simulink model "ParrotMinidroneKeyboardControl"  (R2025b)
settings: Solver=ode3  StartTime=0  StopTime=TFinal  FixedStep=Ts  RelTol=1e-3  EnableMultiTasking=on
values from neighbouring files (symbols this model uses):
  sensorCalibrationData = [0.09 -0.06 -9.473 -0.0095 -0.0075 0.0015 101270.95 0.2]    [sensorCalibration.mat]
undefined symbols (not defined in the file or in its folder): Command, ft, gcbh, init, m, Rec, s, SDTV, Sensors, States, stop_time, takeOffDuration, Ts, Vehicle, vrmfunc, VTs
libraries: simulink x16, aerolibconvert2 x4, SignalEditorBlockLib x2, environmentLibrary x2, visionconversions x2, visiongeotforms x2, aerolibutil x2, aerolibanimutils x1, aerolibnav x1, vrlib x1
(part 1 of 2)
settings Model: ModifiedByFormat=Krishna vamshi challa  ExtModeTrigDuration=80  Creator=The MathWorks, Inc.  LastModifiedBy=Krishna vamshi challa
settings SolverCC: AlgebraicLoopSolver=TrustRegion
settings DataIOCC: LimitDataPoints=on  SaveFormat=Array
settings OptimizationCC: BlockReduction=off  DefaultParameterBehavior=Inlined  EnhancedBackFolding=on  PassReuseOutputArgsAs=Individual arguments  ZeroExternalMemoryAtStartup=off  ZeroInternalMemoryAtStartup=off  MaxStackSize=64  OptimizeBlockOrder=speed  DifferentSizesBufferReuse=on  OptimizationCustomize=off  EfficientTunableParamExpr=on
settings DebuggingCC: AlgebraicLoopMsg=none  ParameterPrecisionLossMsg=none  ParameterTunabilityLossMsg=error  AllowSymbolicDim=off  PregeneratedLibrarySubsystemCodeDiagnostic=none  SubsystemReferenceDiagnosticForUnitTest=warning  SFUnexpectedBacktrackingDiag=warning  SFNoUnconditionalDefaultTransitionDiag=warning  SFExecutionAtInitializationDiag=none  ArithmeticOperatorsInVariantConditions=warning
settings HardwareCC: ProdBitPerPointer=32.0  ProdBitPerSizeT=32.0  ProdBitPerPtrDiffT=32.0  ProdLargestAtomicInteger=Long  ProdWordSize=32.0  ProdHWDeviceType=ARM Compatible->ARM 9
settings ModelReferenceCC: EnableRefExpFcnMdlSchedulingChecks=on  PropagateSignalLabelsOutOfModel=off
settings SFSimCC: SimUseLocalCustomCode=off  MATLABDynamicMemAlloc=off
settings RTWCC: SystemTargetFile=ert.tlc  HardwareBoard=PARROT Mambo  TemplateMakefile=ert_default_tmf  GenerateReport=on  RTWUseLocalCustomCode=off  Toolchain=Sourcery G++ Lite GNU Toolchain for Drones  LaunchReport=on  TargetLang=C++  GPUComputeCapability=3.5  Description=Embedded Coder
settings CodeAppCC: ForceParamTrailComments=on  IgnoreCustomStorageClasses=off  OperatorAnnotations=on  SimulinkDataObjDesc=on  SFDataObjDesc=on  InsertBlockDesc=on
settings ERTTargetCC: ExtModeMaxTrigDuration=80.0  RootIOFormat=Structure reference  TargetLangStandard=C++11 (ISO)  CodeInterfacePackaging=C++ class  SubcomponentCodeInterfacePackaging=C++ class
settings ConfigComp: CovMetricSettings=dw  CovSaveCumulativeToWorkspaceVar=on  CovSaveSingleToWorkspaceVar=on  CovExternalEMLEnable=off  CovSFcnEnable=off

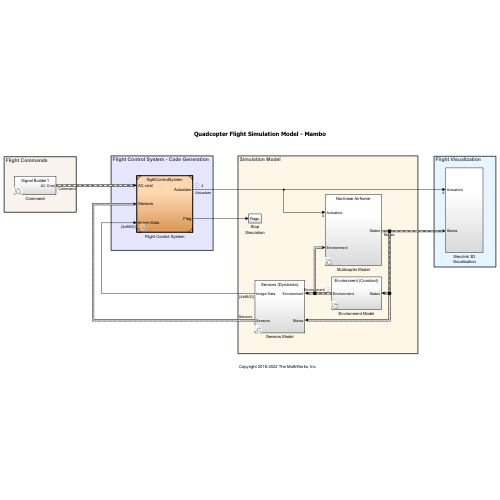
[thumbnail: Simulink's stored preview of the top-level diagram]
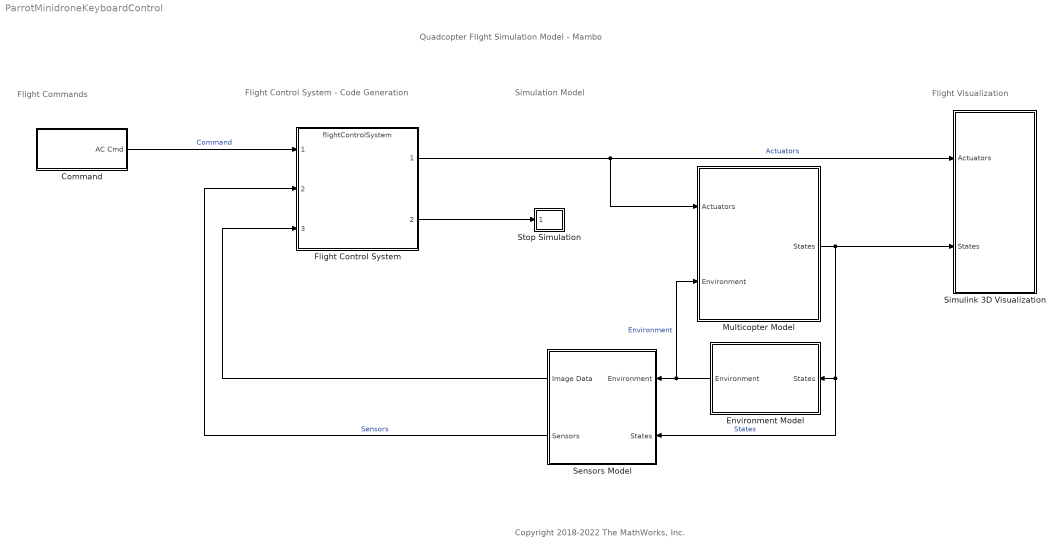
== system ParrotMinidroneKeyboardControl ==
  note: Flight Visualization
  note: Simulation Model
  note: Flight Control System - Code Generation
  note: Flight Commands
  note: Quadcopter Flight Simulation Model - Mambo
  note: Copyright 2018-2022 The MathWorks, Inc.
  Command : Subsystem  Variant=on
  Environment Model : Subsystem  Variant=on
  Flight Control System : ModelReference  ModelNameDialog=flightControlSystem.slx  SimulationMode=Normal  ModelReferenceVersion=11.6
  Multicopter Model : Subsystem  Variant=on
  Sensors Model : Subsystem  Variant=on
  Simulink 3D Visualization : Subsystem
  Stop Simulation : Subsystem
  wires:
  Command/1(AC Cmd) -> Flight Control System/1  "Command"
  Sensors Model/2(Sensors) -> Flight Control System/2  "Sensors"
  Flight Control System/1 -> Multicopter Model/1(Actuators), Simulink 3D Visualization/1(Actuators)  "Actuators"
  Environment Model/1(Environment) -> Sensors Model/1(Environment), Multicopter Model/2(Environment)  "Environment"
  Multicopter Model/1(States) -> Sensors Model/2(States), Environment Model/1(States), Simulink 3D Visualization/2(States)  "States"
  Flight Control System/2 -> Stop Simulation/1(Flags)
  Sensors Model/1(Image Data) -> Flight Control System/3

== system ParrotMinidroneKeyboardControl/Command ==
  note: VSS_COMMAND = 0 will select Signal Builder
      | VSS_COMMAND =1 will select Joystick + Signal Builder
      | VSS_COMMAND = 2 will select pre-saved data from .mat file
      | VSS_COMMAND = 3 will select pre-saved data from a spreadsheet
  Data : Subsystem  VariantControl=VSS_COMMAND_PRESAVED
  Joystick : Subsystem  VariantControl=VSS_COMMAND_JOYSTICK
  Signal Builder1 : Subsystem  VariantControl=VSS_COMMAND_SIGBLDR
  Spreadsheet Data : Subsystem  VariantControl=VSS_COMMAND_SPREADSHEET
  AC Cmd : Outport  OutDataTypeStr=Bus: CommandBus  VectorParamsAs1DForOutWhenUnconnected=off

== system ParrotMinidroneKeyboardControl/Environment Model ==
  note: VSS_ENVIRONMENT = 0 will select constant environment variables
      | VSS_ENVIRONMENT = 1 will select environment variables depending on position
  States : Inport  OutDataTypeStr=Bus: StatesBus
  Environment (Constant) : environmentLibrary/Environment (Constant)  SystemSampleTime=-1  VariantControl=VSS_ENVIRONMENT_CST  VariantActivationTime=update diagram  EmptyChoice=off  PassThrough=off  PassThroughVariantControl=(default)  EmptyChoiceVariantControl=(default)  AllowFlexibleInterface=on  Latency=0  AutoFrameSizeCalculation=off
  Environment (Variable) : environmentLibrary/Environment (Variable)  SystemSampleTime=-1  VariantControl=VSS_ENVIRONMENT_VARIABLE  VariantActivationTime=update diagram  AllowFlexibleInterface=on  Latency=0  AutoFrameSizeCalculation=off
  Environment : Outport  OutDataTypeStr=Bus: EnvironmentBus  VectorParamsAs1DForOutWhenUnconnected=off

== system ParrotMinidroneKeyboardControl/Multicopter Model ==
  note: VSS_VEHICLE = 0 will select linear airframe
      | VSS_VEHICLE = 1 will select nonlnear airframe
  Actuators : Inport
  Environment : Inport  Port=2  OutDataTypeStr=Bus: EnvironmentBus
  Linear Airframe : ModelReference  ModelNameDialog=linearAirframe.slx  SimulationMode=Normal  VariantControl=VSS_VEHICLE_LINEAR  ModelReferenceVersion=10.0
  Nonlinear Airframe : ModelReference  ModelNameDialog=nonlinearAirframe.slx  SimulationMode=Normal  VariantControl=VSS_VEHICLE_NONLINEAR  ModelReferenceVersion=12.2
  States : Outport  OutDataTypeStr=Bus: StatesBus  VectorParamsAs1DForOutWhenUnconnected=off

== system ParrotMinidroneKeyboardControl/Sensors Model ==
  note: VSS_SENSORS = 0 will select feedthrough sensors
      | VSS_SENSORS = 1 will select dynamics sensors with noise
  Environment : Inport
  States : Inport  Port=2
  Sensors (Dynamics) : Subsystem  TreatAsAtomicUnit=on  VariantControl=VSS_SENSORS_DYNAMICS
  Sensors (Feedthrough) : Subsystem  TreatAsAtomicUnit=on  VariantControl=VSS_SENSORS_FEEDTHROUGH
  Image Data : Outport  VectorParamsAs1DForOutWhenUnconnected=off
  Sensors : Outport  Port=2  VectorParamsAs1DForOutWhenUnconnected=off

== system ParrotMinidroneKeyboardControl/Simulink 3D Visualization ==
  Actuators : Inport
  States : Inport  Port=2
  Airspeed Indicator : AirspeedIndicatorBlock  LabelPosition=Hide
  Altimeter : AltimeterBlock  LabelPosition=Hide
  Artificial Horizon : ArtificialHorizonBlock  LabelPosition=Hide
  Climb Rate Indicator : ClimbIndicatorBlock  LabelPosition=Hide
  Extract Flight Instruments : Subsystem
  Heading Indicator1 : HeadingIndicatorBlock  LabelPosition=Hide
  Simulink 3D : Subsystem  VariantControl=VSS_VISUALIZATION_SL3D
      mask init:
      | visualizationFlightGearVars;
  Thruster {1..4} (4 alike) : RPMIndicatorBlock  LabelPosition=Hide
  wires:
  Actuators/1 -> Extract Flight Instruments/1(Actuators), Simulink 3D/2(Actuators)
  States/1 -> Extract Flight Instruments/2(States), Simulink 3D/1(States)

== system ParrotMinidroneKeyboardControl/Stop Simulation ==
  Flags : Inport  OutDataTypeStr=uint8
  Compare To Zero : simulink/Logic and Bit Operations/Compare To Zero  relop=>  OutDataTypeStr=boolean
  Flag has been triggered : Assertion
  Logical Operator : Logic  Operator=NOT  AllPortsSameDT=off  OutDataTypeStr=boolean
  wires:
  Flags/1 -> Compare To Zero/1
  Logical Operator/1 -> Flag has been triggered/1
  Compare To Zero/1 -> Logical Operator/1

== system ParrotMinidroneKeyboardControl/Command/Data ==
  Bus Creator : BusCreator  Inputs=5  OutDataTypeStr=Bus: CommandBus  NonVirtualBus=on
  Clock : Clock
  Compare To Constant : simulink/Logic and Bit Operations/Compare To Constant  relop=<  const=takeOffDuration  OutDataTypeStr=boolean
  Compare To Zero : simulink/Logic and Bit Operations/Compare To Zero  relop===  OutDataTypeStr=boolean
  Compare To Zero1 : simulink/Logic and Bit Operations/Compare To Zero  relop===  OutDataTypeStr=boolean
  Data Type Conversion1 : DataTypeConversion  OutDataTypeStr=single  SaturateOnIntegerOverflow=off  RndMeth=Floor
  Data Type Conversion3 : DataTypeConversion  OutDataTypeStr=single  SaturateOnIntegerOverflow=off  RndMeth=Floor
  Demux : Demux  Outputs=6
  From File : FromFile  FileName=cmdData.mat  SampleTime=Ts
  Live Time Ticks : simulink/Sources/Counter Free-Running  NumBits=32  tsamp=Ts
  Logical Operator : Logic  AllPortsSameDT=off  OutDataTypeStr=boolean
  Mux : Mux  Inputs=3
  Mux1 : Mux  Inputs=3
  Rate Transition{1..4} (4 alike) : RateTransition  OutPortSampleTime=Ts
  AC Cmd : Outport  OutDataTypeStr=Bus: CommandBus  VectorParamsAs1DForOutWhenUnconnected=off
  wires:
  Demux/4 -> Mux/1  "roll_cmd"
  Demux/5 -> Mux/2, Compare To Zero1/1  "pitch_cmd"
  Demux/6 -> Compare To Zero/1, Mux/3  "yaw_cmd"
  From File/1 -> Demux/1
  Logical Operator/1 -> Rate Transition4/1
  Rate Transition1/1 -> Bus Creator/4  "orient_ref"
  Rate Transition2/1 -> Bus Creator/2  "pos_ref"
  Demux/3 -> Mux1/3
  Mux/1 -> Data Type Conversion3/1
  Data Type Conversion1/1 -> Rate Transition2/1
  Demux/1 -> Mux1/1
  Compare To Zero1/1 -> Logical Operator/2
  Compare To Zero/1 -> Logical Operator/1
  Mux1/1 -> Data Type Conversion1/1
  Clock/1 -> Compare To Constant/1
  Rate Transition4/1 -> Bus Creator/1  "controlModePosVSOrient"
  Data Type Conversion3/1 -> Rate Transition1/1
  Demux/2 -> Mux1/2
  Compare To Constant/1 -> Rate Transition3/1
  Rate Transition3/1 -> Bus Creator/3  "takeoff_flag"
  Live Time Ticks/1 -> Bus Creator/5  "live_time_ticks"
  Bus Creator/1 -> AC Cmd/1

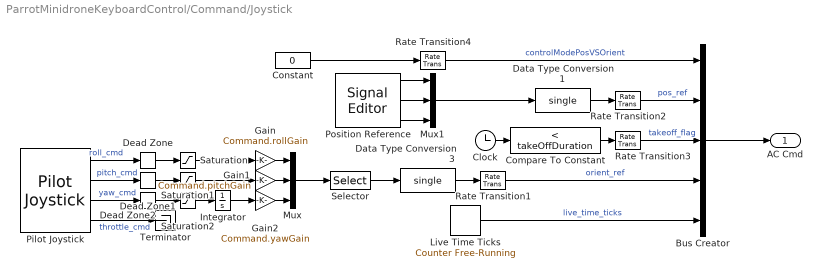
== system ParrotMinidroneKeyboardControl/Command/Joystick ==
  Bus Creator : BusCreator  Inputs=5  OutDataTypeStr=Bus: CommandBus  NonVirtualBus=on
  Clock : Clock
  Compare To Constant : simulink/Logic and Bit Operations/Compare To Constant  relop=<  const=takeOffDuration  OutDataTypeStr=boolean
  Constant : Constant  Value=0  OutDataTypeStr=boolean
  Data Type Conversion1 : DataTypeConversion  OutDataTypeStr=single  SaturateOnIntegerOverflow=off  RndMeth=Floor
  Data Type Conversion3 : DataTypeConversion  OutDataTypeStr=single  SaturateOnIntegerOverflow=off  RndMeth=Floor
  Dead Zone : DeadZone  LowerValue=Command.rollDeadZoneStart  UpperValue=Command.rollDeadZoneEnd
  Dead Zone1 : DeadZone  LowerValue=Command.pitchDeadZoneStart  UpperValue=Command.pitchDeadZoneEnd
  Dead Zone2 : DeadZone  LowerValue=Command.yawDeadZoneStart  UpperValue=Command.yawDeadZoneEnd
  Gain : Gain  Gain=Command.rollGain
  Gain1 : Gain  Gain=Command.pitchGain
  Gain2 : Gain  Gain=Command.yawGain
  Integrator : Integrator
  Live Time Ticks : simulink/Sources/Counter Free-Running  NumBits=32  tsamp=Ts
  Mux : Mux  Inputs=3
  Mux1 : Mux  Inputs=3
  Pilot Joystick : aerolibanimutils/Pilot Joystick  JoystickID=Joystick1  OutputConfiguration=FourAxis  SampleTime=Ts
  Position Reference : SignalEditorBlockLib/Signal Editor  FileName=Position_Reference.mat  ActiveScenario=Group_1  ActiveSignal=Z  IsBus=off  OutputBusObjectStr=Bus: BusObject  SampleTime=0  OutputAfterFinalValue=Extrapolation  Unit=inherit  PreserveSignalName=on  ApplySigPropsToAllScenarios=on  ApplySigPropsToAllSignals=off
  Rate Transition{1..4} (4 alike) : RateTransition  OutPortSampleTime=Ts
  Saturation : Saturate  UpperLimit=Command.rollSatUpper  LowerLimit=Command.rollSatLower
  Saturation1 : Saturate  UpperLimit=Command.pitchSatUpper  LowerLimit=Command.pitchSatLower
  Saturation2 : Saturate  UpperLimit=Command.yawSatUpper  LowerLimit=Command.yawSatLower
  Selector : Selector  InputPortWidth=3  IndexOptions=Index vector (dialog)  Indices=[3 2 1]  OutputSizes=1
  Terminator : Terminator
  AC Cmd : Outport  OutDataTypeStr=Bus: CommandBus  VectorParamsAs1DForOutWhenUnconnected=off
  wires:
  Pilot Joystick/4 -> Terminator/1  "throttle_cmd"
  Pilot Joystick/1 -> Dead Zone/1  "roll_cmd"
  Bus Creator/1 -> AC Cmd/1
  Constant/1 -> Rate Transition4/1
  Rate Transition1/1 -> Bus Creator/4  "orient_ref"
  Rate Transition2/1 -> Bus Creator/2  "pos_ref"
  Position Reference/3 -> Mux1/3
  Mux/1 -> Selector/1
  Data Type Conversion1/1 -> Rate Transition2/1
  Position Reference/1 -> Mux1/1
  Mux1/1 -> Data Type Conversion1/1
  Compare To Constant/1 -> Rate Transition3/1
  Clock/1 -> Compare To Constant/1
  Rate Transition4/1 -> Bus Creator/1  "controlModePosVSOrient"
  Data Type Conversion3/1 -> Rate Transition1/1
  Pilot Joystick/2 -> Dead Zone1/1  "pitch_cmd"
  Position Reference/2 -> Mux1/2
  Rate Transition3/1 -> Bus Creator/3  "takeoff_flag"
  Live Time Ticks/1 -> Bus Creator/5  "live_time_ticks"
  Selector/1 -> Data Type Conversion3/1
  Dead Zone/1 -> Saturation/1
  Saturation/1 -> Gain/1
  Gain/1 -> Mux/1
  Dead Zone1/1 -> Saturation1/1
  Saturation1/1 -> Gain1/1
  Gain1/1 -> Mux/2
  Dead Zone2/1 -> Saturation2/1
  Saturation2/1 -> Integrator/1
  Gain2/1 -> Mux/3
  Pilot Joystick/3 -> Dead Zone2/1  "yaw_cmd"
  Integrator/1 -> Gain2/1

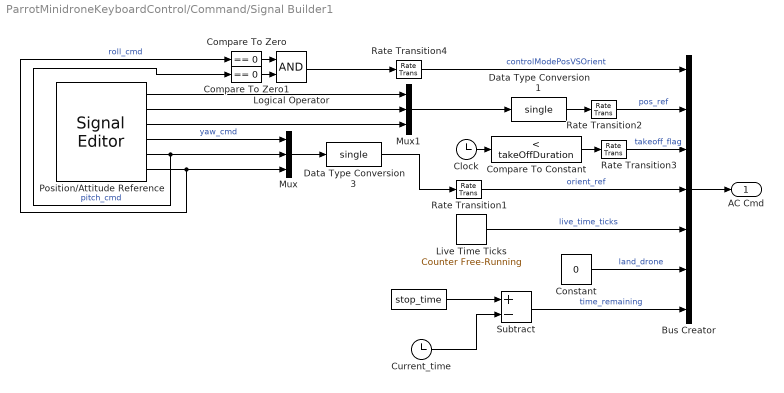
== system ParrotMinidroneKeyboardControl/Command/Signal Builder1 ==
  " " : Constant  InitFcn=|  Value=stop_time
      | sim_model = split(gcs,"/");
      | stop_time_str = get_param(sim_model{1},'stopTime');
      | stop_time = evalin('base', stop_time_str);
      settings: DeleteFcn=clear sim_model stop_time_str stop_time
  Bus Creator : BusCreator  Inputs=7  OutDataTypeStr=Bus: CommandBus  NonVirtualBus=on
  Clock : Clock
  Compare To Constant : simulink/Logic and Bit Operations/Compare To Constant  relop=<  const=takeOffDuration  OutDataTypeStr=boolean
  Compare To Zero : simulink/Logic and Bit Operations/Compare To Zero  relop===  OutDataTypeStr=boolean
  Compare To Zero1 : simulink/Logic and Bit Operations/Compare To Zero  relop===  OutDataTypeStr=boolean
  Constant : Constant  Value=0  OutDataTypeStr=boolean
  Current_time : Clock
  Data Type Conversion1 : DataTypeConversion  OutDataTypeStr=single  SaturateOnIntegerOverflow=off  RndMeth=Floor
  Data Type Conversion3 : DataTypeConversion  OutDataTypeStr=single  SaturateOnIntegerOverflow=off  RndMeth=Floor
  Live Time Ticks : simulink/Sources/Counter Free-Running  NumBits=32  tsamp=Ts
  Logical Operator : Logic  AllPortsSameDT=off  OutDataTypeStr=boolean
  Mux : Mux  Inputs=3
  Mux1 : Mux  Inputs=3
  Position/Attitude Reference : SignalEditorBlockLib/Signal Editor  FileName=Position_Attitude_Reference.mat  ActiveScenario=Group_1  ActiveSignal=Roll  IsBus=off  OutputBusObjectStr=Bus: BusObject  SampleTime=0  OutputAfterFinalValue=Extrapolation  Unit=inherit  PreserveSignalName=on  ApplySigPropsToAllScenarios=on  ApplySigPropsToAllSignals=off  SignalPropertySource=Dialog parameters
  Rate Transition{1..4} (4 alike) : RateTransition  OutPortSampleTime=Ts
  Subtract : Sum  Inputs=+-
  AC Cmd : Outport  OutDataTypeStr=Bus: CommandBus  VectorParamsAs1DForOutWhenUnconnected=off
  wires:
  Bus Creator/1 -> AC Cmd/1
  Position/Attitude Reference/6 -> Compare To Zero/1, Mux/3  "roll_cmd"
  Position/Attitude Reference/5 -> Mux/2, Compare To Zero1/1  "pitch_cmd"
  Position/Attitude Reference/4 -> Mux/1  "yaw_cmd"
  Mux/1 -> Data Type Conversion3/1
  Data Type Conversion3/1 -> Rate Transition1/1
  Rate Transition1/1 -> Bus Creator/4  "orient_ref"
  Compare To Zero/1 -> Logical Operator/1
  Compare To Zero1/1 -> Logical Operator/2
  Logical Operator/1 -> Rate Transition4/1
  Rate Transition4/1 -> Bus Creator/1  "controlModePosVSOrient"
  Position/Attitude Reference/1 -> Mux1/1
  Position/Attitude Reference/2 -> Mux1/2
  Position/Attitude Reference/3 -> Mux1/3
  Mux1/1 -> Data Type Conversion1/1
  Data Type Conversion1/1 -> Rate Transition2/1
  Rate Transition2/1 -> Bus Creator/2  "pos_ref"
  Clock/1 -> Compare To Constant/1
  Compare To Constant/1 -> Rate Transition3/1
  Rate Transition3/1 -> Bus Creator/3  "takeoff_flag"
  Live Time Ticks/1 -> Bus Creator/5  "live_time_ticks"
  Constant/1 -> Bus Creator/6  "land_drone"
  Subtract/1 -> Bus Creator/7  "time_remaining"
  Current_time/1 -> Subtract/2
  " "/1 -> Subtract/1

== system ParrotMinidroneKeyboardControl/Command/Spreadsheet Data ==
  Bus Creator : BusCreator  Inputs=5  OutDataTypeStr=Bus: CommandBus  NonVirtualBus=on
  Clock : Clock
  Compare To Constant : simulink/Logic and Bit Operations/Compare To Constant  relop=<  const=takeOffDuration  OutDataTypeStr=boolean
  Compare To Zero : simulink/Logic and Bit Operations/Compare To Zero  relop===  OutDataTypeStr=boolean
  Compare To Zero1 : simulink/Logic and Bit Operations/Compare To Zero  relop===  OutDataTypeStr=boolean
  Data Type Conversion1 : DataTypeConversion  OutDataTypeStr=single  SaturateOnIntegerOverflow=off  RndMeth=Floor
  Data Type Conversion3 : DataTypeConversion  OutDataTypeStr=single  SaturateOnIntegerOverflow=off  RndMeth=Floor
  From Spreadsheet : FromSpreadsheet  FileName=cmdData.xlsx  SheetName=data  SampleTime=Ts
  Live Time Ticks : simulink/Sources/Counter Free-Running  NumBits=32  tsamp=Ts
  Logical Operator : Logic  AllPortsSameDT=off  OutDataTypeStr=boolean
  Mux : Mux  Inputs=3
  Mux1 : Mux  Inputs=3
  Rate Transition{1..4} (4 alike) : RateTransition  OutPortSampleTime=Ts
  AC Cmd : Outport  OutDataTypeStr=Bus: CommandBus  VectorParamsAs1DForOutWhenUnconnected=off
  wires:
  Bus Creator/1 -> AC Cmd/1
  From Spreadsheet/4 -> Mux/1  "roll_cmd"
  From Spreadsheet/6 -> Mux/3, Compare To Zero/1  "yaw_cmd"
  Logical Operator/1 -> Rate Transition4/1
  Rate Transition1/1 -> Bus Creator/4  "orient_ref"
  Rate Transition2/1 -> Bus Creator/2  "pos_ref"
  From Spreadsheet/3 -> Mux1/3
  Mux/1 -> Data Type Conversion3/1
  Data Type Conversion1/1 -> Rate Transition2/1
  From Spreadsheet/1 -> Mux1/1
  Compare To Zero1/1 -> Logical Operator/2
  Compare To Zero/1 -> Logical Operator/1
  Mux1/1 -> Data Type Conversion1/1
  Compare To Constant/1 -> Rate Transition3/1
  Clock/1 -> Compare To Constant/1
  Rate Transition4/1 -> Bus Creator/1  "controlModePosVSOrient"
  Data Type Conversion3/1 -> Rate Transition1/1
  From Spreadsheet/5 -> Mux/2, Compare To Zero1/1  "pitch_cmd"
  From Spreadsheet/2 -> Mux1/2
  Rate Transition3/1 -> Bus Creator/3  "takeoff_flag"
  Live Time Ticks/1 -> Bus Creator/5  "live_time_ticks"

== system ParrotMinidroneKeyboardControl/Sensors Model/Sensors (Dynamics) ==
  States : Inport  OutDataTypeStr=Bus: StatesBus
  Environment : Inport  Port=2  OutDataTypeStr=Bus: EnvironmentBus
  Bus Creator1 : BusCreator  Inputs=3  OutDataTypeStr=Bus: SensorsBus  NonVirtualBus=on
  Bus Creator2 : BusCreator  Inputs=3  OutDataTypeStr=Bus: extraSensorData_t  NonVirtualBus=on
  Constant : Constant  Value=sensorCalibrationData  OutDataTypeStr=single
  Memory1 : Memory  InitialCondition=States  InheritSampleTime=on
  Sensor System : Subsystem
  _DUMMY_FLAG_usePosVIS : Constant  Value=Sensors.dummy.usePosVISFlag  OutDataTypeStr=single  SampleTime=Ts
  _DUMMY_posVIS : Constant  Value=Sensors.dummy.posVISNoVisionAvail  OutDataTypeStr=single  SampleTime=Ts
  Sensors : Outport  OutDataTypeStr=Bus: SensorsBus  VectorParamsAs1DForOutWhenUnconnected=off
  Image Data : Outport  Port=2  VectorParamsAs1DForOutWhenUnconnected=off
  wires:
  Constant/1 -> Bus Creator1/3  "SensorCalibration"
  Memory1/1 -> Sensor System/1(States)
  Bus Creator2/1 -> Bus Creator1/1  "VisionSensors"
  Bus Creator1/1 -> Sensors/1
  States/1 -> Memory1/1
  Environment/1 -> Sensor System/2(Environment)
  _DUMMY_FLAG_usePosVIS/1 -> Bus Creator2/3  "usePosVIS_flag"
  _DUMMY_posVIS/1 -> Bus Creator2/2  "posVIS_data"
  Sensor System/1(opticalFlow_data) -> Bus Creator2/1  "opticalFlow_data"
  Sensor System/2(sensordata_data) -> Bus Creator1/2  "HALSensors"
  Sensor System/3(camera_data) -> Image Data/1

== system ParrotMinidroneKeyboardControl/Sensors Model/Sensors (Feedthrough) ==
  States : Inport  OutDataTypeStr=Bus: StatesBus
  Environment : Inport  Port=2  OutDataTypeStr=Bus: EnvironmentBus
  Bus Creator1 : BusCreator  Inputs=3  OutDataTypeStr=Bus: SensorsBus  NonVirtualBus=on
  Bus Creator2 : BusCreator  Inputs=3  OutDataTypeStr=Bus: extraSensorData_t  NonVirtualBus=on
  Constant1 : Constant  Value=sensorCalibrationData  OutDataTypeStr=single
  Memory : Memory  InitialCondition=States  InheritSampleTime=on
  Sensor System : Subsystem
  _DUMMY_FLAG_usePosVIS : Constant  Value=Sensors.dummy.usePosVISFlag  OutDataTypeStr=single
  _DUMMY_posVIS : Constant  Value=Sensors.dummy.posVISNoVisionAvail  OutDataTypeStr=single
  Sensors : Outport  OutDataTypeStr=Bus: SensorsBus  VectorParamsAs1DForOutWhenUnconnected=off
  Image Data : Outport  Port=2  VectorParamsAs1DForOutWhenUnconnected=off
  wires:
  Constant1/1 -> Bus Creator1/3  "SensorCalibration"
  Memory/1 -> Sensor System/1(States)
  Sensor System/2(sensordata_data) -> Bus Creator1/2  "HALSensors"
  States/1 -> Memory/1
  Environment/1 -> Sensor System/2(Environment)
  Bus Creator1/1 -> Sensors/1
  _DUMMY_FLAG_usePosVIS/1 -> Bus Creator2/3  "usePosVIS_flag"
  Sensor System/1(opticalFlow_data) -> Bus Creator2/1  "opticalFlow_data"
  _DUMMY_posVIS/1 -> Bus Creator2/2  "posVIS_data"
  Bus Creator2/1 -> Bus Creator1/1  "VisionSensors"
  Sensor System/3(camera_data) -> Image Data/1

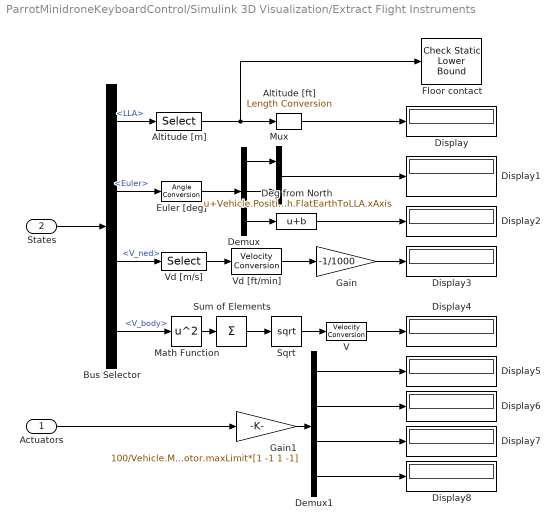
== system ParrotMinidroneKeyboardControl/Simulink 3D Visualization/Extract Flight Instruments ==
  Actuators : Inport
  States : Inport  Port=2
  Altitude [ft] : aerolibconvert2/Length Conversion  IU=m  OU=ft
  Altitude [m] : Selector  InputPortWidth=3  IndexOptions=Index vector (dialog)  Indices=[3]  OutputSizes=1
  Bus Selector : BusSelector  OutputSignals=LLA,Euler,V_ned,V_body
  Deg from North : Bias  Bias=Vehicle.PositionOnEarth.FlatEarthToLLA.xAxis  SaturateOnIntegerOverflow=off
  Demux : Demux  Outputs=3
  Demux1 : Demux
  Display{,1..8} (9 alike) : Display
  Euler [deg] : aerolibconvert2/Angle Conversion  IU=rad  OU=deg
  Floor contact : simulink/Model Verification/Check Static  Lower Bound  Description=init.posLLA(3) <= u  min=init.posLLA(3)  min_included=on  enabled=on  stopWhenAssertionFail=on  export=off  icon=graphic
  Gain : Gain  Gain=-1/1000
  Gain1 : Gain  Gain=100/Vehicle.Motor.maxLimit*[1 -1 1 -1]
  Math Function : Math  Operator=square  SignedPower=on
  Mux : Mux  Inputs=2
  Sqrt : Sqrt
  Sum of Elements : Sum  Inputs=+
  V : aerolibconvert2/Velocity Conversion  IU=m/s  OU=kts
  Vd [ft/min] : aerolibconvert2/Velocity Conversion  IU=m/s  OU=ft/min
  Vd [m/s] : Selector  InputPortWidth=3  IndexOptions=Index vector (dialog)  Indices=[3]  OutputSizes=1
  wires:
  Bus Selector/1 -> Altitude [m]/1  "<LLA>"
  Altitude [m]/1 -> Floor contact/1, Altitude [ft]/1
  States/1 -> Bus Selector/1
  Altitude [ft]/1 -> Display/1
  Bus Selector/2 -> Euler [deg]/1  "<Euler>"
  Euler [deg]/1 -> Demux/1
  Demux/1 -> Mux/1
  Demux/2 -> Mux/2
  Mux/1 -> Display1/1
  Deg from North/1 -> Display2/1
  Bus Selector/3 -> Vd [m/s]/1  "<V_ned>"
  Vd [m/s]/1 -> Vd [ft/min]/1
  Vd [ft/min]/1 -> Gain/1
  Gain/1 -> Display3/1
  Math Function/1 -> Sum of Elements/1
  Sum of Elements/1 -> Sqrt/1
  Bus Selector/4 -> Math Function/1  "<V_body>"
  Sqrt/1 -> V/1
  V/1 -> Display4/1
  Gain1/1 -> Demux1/1
  Demux1/1 -> Display5/1
  Demux1/2 -> Display6/1
  Demux1/3 -> Display7/1
  Demux1/4 -> Display8/1
  Actuators/1 -> Gain1/1
  Demux/3 -> Deg from North/1

== system ParrotMinidroneKeyboardControl/Simulink 3D Visualization/Simulink 3D ==
  States : Inport
  Actuators : Inport  Port=2
  Axes to VR Axes : Subsystem
  Axes to VR Axes Camera Chase : Subsystem
  Axes to VR Axes Camera Iso : Subsystem
  Bus Selector : BusSelector  OutputSignals=Euler,X_ned
  Camera bias Chase : Bias  Bias=[-4 0 -.9558]'  SaturateOnIntegerOverflow=off
  Camera bias Iso : Bias  Bias=[0.9009 .99 -.6247]'  SaturateOnIntegerOverflow=off
  Euler to VR : Subsystem
  Rate Transition{,1..3} (4 alike) : RateTransition
  Subsystem : Subsystem
  VR Sink : vrlib/VR Sink  InstantiateOnLoad=on  SampleTime=12*Ts  ViewEnable=on  RemoteChange=off  RemoteView=off  FieldsWritten=QuadBody.rotation.4.1.1.double#QuadBody.translation.3.1.1.double#Blade1.rotation.4.1.1.double#Blade3.rotation.4.1.1.double#Blade2.rotation.4.1.1.double#Blade4.rotation.4.1.1.double#IsoNoRotation.position.3.1.1.double#OnQuadNoRotation.position.3.1.1.double  WorldFileName=asbQuadcopterWorld.wrl  WorldDescription=Minidrone Flight Visualization  AutoView=on  VideoDimensions=[]  AllowVariableSize=off  FigureProperties="{'Position', 'Name', 'Viewpoint', 'CameraBound', 'CameraDirection', 'CameraPosition', 'CameraUpVector', 'ZoomFactor', 'Antialiasing', 'Headlight', 'Lighting', 'Sound', 'StatusBar', 'Stereo3D', 'Stereo3DCameraOffset', 'Stereo3DHIT', 'ToolBar', 'Textures', 'Transparency', 'Triad', 'Wireframe', 'NavZones', 'NavMode', 'NavSpeed', 'CaptureFileFormat', 'CaptureFileName', 'Record2DCompressMethod', 'Record2DCompressQuality', 'Record2D', 'Record2DFileName', 'Record2DFPS'; [5.0000000000000000e+00   9.2000000000000000e+01   5.7600000000000000e+02   3.8000000000000000e+02], 'Minidrone Flight Visualization', 'Isometric', 'on', [0.0000000000000000e+00   0.0000000000000000e+00  -1.0000000000000000e+00], [0.0000000000000000e+00   0.0000000000000000e+00   0.0000000000000000e+00], [0.0000000000000000e+00   1.0000000000000000e+00   0.0000000000000000e+00], [1.0000000000000000e+00], 'on', 'on', 'on', 'off', 'on', 'off', [1.0000000000000001e-01], [0.0000000000000000e+00], 'on', 'on', 'on', 'none', 'off', 'off', 'examine', 'normal', 'tif', '%f_anim_%n.tif', 'auto', [7.5000000000000000e+01], 'off', '%f_anim_%n.avi', 'auto'}"
  wires:
  Euler to VR/1(Axis Angle) -> Rate Transition/1
  Axes to VR Axes/1(Xe VR) -> Rate Transition1/1
  Bus Selector/1 -> Euler to VR/1(Euler Angles)  "<Euler>"
  Bus Selector/2 -> Camera bias Chase/1, Camera bias Iso/1, Axes to VR Axes/1(Xe)  "<X_ned>"
  States/1 -> Bus Selector/1
  Actuators/1 -> Subsystem/1(Actuators)
  Axes to VR Axes Camera Iso/1(Xe VR) -> Rate Transition2/1
  Camera bias Iso/1 -> Axes to VR Axes Camera Iso/1(Xe)
  Rate Transition/1 -> VR Sink/1
  Rate Transition1/1 -> VR Sink/2
  Subsystem/1(Position Blade1) -> VR Sink/3
  Subsystem/2(Position Blade 2) -> VR Sink/4
  Subsystem/3(Position Blade 3) -> VR Sink/5
  Subsystem/4(Position Blade 4) -> VR Sink/6
  Rate Transition2/1 -> VR Sink/7
  Axes to VR Axes Camera Chase/1(Xe VR) -> Rate Transition3/1
  Rate Transition3/1 -> VR Sink/8
  Camera bias Chase/1 -> Axes to VR Axes Camera Chase/1(Xe)

== system ParrotMinidroneKeyboardControl/Sensors Model/Sensors (Dynamics)/Sensor System ==
  States : Inport
  Environment : Inport  Port=2
  Camera : Subsystem
  IMU_Pressure : Subsystem
  Rate Transition1 : RateTransition  OutPortSampleTime=Ts
  Rate Transition2 : RateTransition  OutPortSampleTime=Ts
  opticalFlow_data : Outport  VectorParamsAs1DForOutWhenUnconnected=off
  sensordata_data : Outport  Port=2  OutDataTypeStr=Bus: HAL_acquisition_t  VectorParamsAs1DForOutWhenUnconnected=off
  camera_data : Outport  Port=3  VectorParamsAs1DForOutWhenUnconnected=off
  wires:
  Environment/1 -> IMU_Pressure/2(Environment)
  Camera/1(opticalFlow_datout) -> Rate Transition1/1
  IMU_Pressure/1(sensordata_datout) -> Rate Transition2/1
  Rate Transition1/1 -> opticalFlow_data/1
  Rate Transition2/1 -> sensordata_data/1
  States/1 -> Camera/1(states), IMU_Pressure/1(States)
  Camera/2(image_data) -> camera_data/1

== system ParrotMinidroneKeyboardControl/Sensors Model/Sensors (Feedthrough)/Sensor System ==
  States : Inport
  Environment : Inport  Port=2
  Camera : Subsystem
  IMU_Pressure : Subsystem
  Rate Transition1 : RateTransition  OutPortSampleTime=Ts
  Rate Transition2 : RateTransition  OutPortSampleTime=Ts
  opticalFlow_data : Outport  VectorParamsAs1DForOutWhenUnconnected=off
  sensordata_data : Outport  Port=2  OutDataTypeStr=Bus: HAL_acquisition_t  VectorParamsAs1DForOutWhenUnconnected=off
  camera_data : Outport  Port=3  VectorParamsAs1DForOutWhenUnconnected=off
  wires:
  Environment/1 -> IMU_Pressure/2(Environment)
  Camera/1(opticalFlow_datout) -> Rate Transition1/1
  IMU_Pressure/1(sensordata_datout) -> Rate Transition2/1
  Rate Transition1/1 -> opticalFlow_data/1
  Rate Transition2/1 -> sensordata_data/1
  States/1 -> Camera/1(states), IMU_Pressure/1(states_datin)
  Camera/2(image_data) -> camera_data/1

== system ParrotMinidroneKeyboardControl/Simulink 3D Visualization/Simulink 3D/Axes to VR Axes ==
  Xe : Inport
  Demux : Demux  Outputs=3
      settings: DisplayOption=none
  Mux : Mux  Inputs=3
  rad-->deg1 : Gain  Gain=-1  SaturateOnIntegerOverflow=on  OutDataTypeStr=Inherit: Same as input  ParamDataTypeStr=Inherit: Same as input
  Xe VR : Outport  VectorParamsAs1DForOutWhenUnconnected=off
  wires:
  Xe/1 -> Demux/1
  Demux/1 -> Mux/1
  Demux/3 -> rad-->deg1/1
  Mux/1 -> Xe VR/1
  rad-->deg1/1 -> Mux/2
  Demux/2 -> Mux/3

== system ParrotMinidroneKeyboardControl/Simulink 3D Visualization/Simulink 3D/Axes to VR Axes Camera Chase ==
  Xe : Inport
  Demux : Demux  Outputs=3
      settings: DisplayOption=none
  Mux : Mux  Inputs=3
  rad-->deg1 : Gain  Gain=-1  SaturateOnIntegerOverflow=on  OutDataTypeStr=Inherit: Same as input  ParamDataTypeStr=Inherit: Same as input
  Xe VR : Outport  VectorParamsAs1DForOutWhenUnconnected=off
  wires:
  Xe/1 -> Demux/1
  Demux/1 -> Mux/1
  Demux/3 -> rad-->deg1/1
  Mux/1 -> Xe VR/1
  rad-->deg1/1 -> Mux/2
  Demux/2 -> Mux/3

== system ParrotMinidroneKeyboardControl/Simulink 3D Visualization/Simulink 3D/Axes to VR Axes Camera Iso ==
  Xe : Inport
  Demux : Demux  Outputs=3
      settings: DisplayOption=none
  Mux : Mux  Inputs=3
  rad-->deg1 : Gain  Gain=-1  SaturateOnIntegerOverflow=on  OutDataTypeStr=Inherit: Same as input  ParamDataTypeStr=Inherit: Same as input
  Xe VR : Outport  VectorParamsAs1DForOutWhenUnconnected=off
  wires:
  Demux/2 -> Mux/3
  rad-->deg1/1 -> Mux/2
  Mux/1 -> Xe VR/1
  Demux/3 -> rad-->deg1/1
  Demux/1 -> Mux/1
  Xe/1 -> Demux/1

== system ParrotMinidroneKeyboardControl/Simulink 3D Visualization/Simulink 3D/Euler to VR ==
  Euler Angles : Inport
  Axis Angle Vector : Subsystem
  Mux : Mux  Inputs=2
  Mux1 : Mux  Inputs=2
  Mux2 : Mux  Inputs=2
  Quaternion Multiplication (Pitch & Yaw) : aerolibutil/Quaternion Multiplication
  Quaternion Multiplication (Roll) : aerolibutil/Quaternion Multiplication
  Quaternion Normalization : Subsystem
  Quaternion Normalization1 : Subsystem
  Quaternion Normalization2 : Subsystem
  Selector : Selector  InputPortWidth=3  IndexOptions=Index vector (dialog)  Indices=[3]  OutputSizes=1
  Selector1 : Selector  InputPortWidth=3  IndexOptions=Index vector (dialog)  Indices=[2]  OutputSizes=1
  Selector2 : Selector  InputPortWidth=3  IndexOptions=Index vector (dialog)  Indices=[1]  OutputSizes=1
  Vr Pitch Axes : Constant  Value=[0 0 1]
  Vr Roll Axes : Constant  Value=[1 0 0]
  Vr Yaw Axes : Constant  Value=[0 -1 0]
  Axis Angle : Outport  VectorParamsAs1DForOutWhenUnconnected=off
  wires:
  Quaternion Multiplication (Roll)/1 -> Axis Angle Vector/1(e0)
  Axis Angle Vector/1(e0_norm) -> Axis Angle/1
  Quaternion Normalization/1(e0_norm) -> Quaternion Multiplication (Roll)/2
  Quaternion Normalization2/1(e0_norm) -> Quaternion Multiplication (Pitch & Yaw)/1
  Quaternion Normalization1/1(e0_norm) -> Quaternion Multiplication (Pitch & Yaw)/2
  Mux2/1 -> Quaternion Normalization2/1(e0)
  Mux1/1 -> Quaternion Normalization1/1(e0)
  Mux/1 -> Quaternion Normalization/1(e0)
  Selector/1 -> Mux2/1
  Vr Yaw Axes/1 -> Mux2/2
  Selector1/1 -> Mux1/1
  Vr Pitch Axes/1 -> Mux1/2
  Selector2/1 -> Mux/1
  Vr Roll Axes/1 -> Mux/2
  Euler Angles/1 -> Selector2/1, Selector1/1, Selector/1
  Quaternion Multiplication (Pitch & Yaw)/1 -> Quaternion Multiplication (Roll)/1

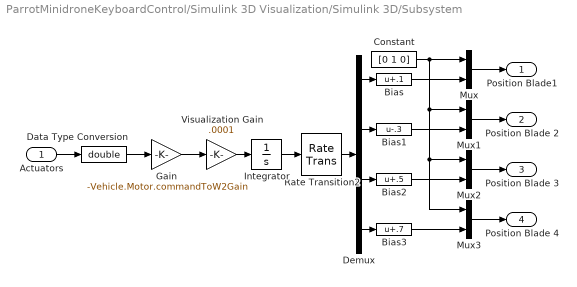
== system ParrotMinidroneKeyboardControl/Simulink 3D Visualization/Simulink 3D/Subsystem ==
  Actuators : Inport
  Bias : Bias  Bias=.1  SaturateOnIntegerOverflow=off
  Bias1 : Bias  Bias=-.3  SaturateOnIntegerOverflow=off
  Bias2 : Bias  Bias=.5  SaturateOnIntegerOverflow=off
  Bias3 : Bias  Bias=.7  SaturateOnIntegerOverflow=off
  Constant : Constant  Value=[0 1 0]
  Data Type Conversion : DataTypeConversion  OutDataTypeStr=double  SaturateOnIntegerOverflow=off  RndMeth=Floor
  Demux : Demux
  Gain : Gain  Gain=-Vehicle.Motor.commandToW2Gain
  Integrator : Integrator  InitialCondition="[.1  .2 -.3 -.4]"  WrapState=on  WrappedStateUpperValue=2*pi  WrappedStateLowerValue=-2*pi
  Mux{,1..3} (4 alike) : Mux  Inputs=2
  Rate Transition2 : RateTransition
  Visualization Gain : Gain  Gain=.0001
  Position Blade1 : Outport  VectorParamsAs1DForOutWhenUnconnected=off
  Position Blade 2 : Outport  Port=2  VectorParamsAs1DForOutWhenUnconnected=off
  Position Blade 3 : Outport  Port=3  VectorParamsAs1DForOutWhenUnconnected=off
  Position Blade 4 : Outport  Port=4  VectorParamsAs1DForOutWhenUnconnected=off
  wires:
  Bias3/1 -> Mux3/2
  Mux3/1 -> Position Blade 4/1
  Bias1/1 -> Mux1/2
  Bias2/1 -> Mux2/2
  Demux/2 -> Bias1/1
  Visualization Gain/1 -> Integrator/1
  Constant/1 -> Mux3/1, Mux2/1, Mux1/1, Mux/1
  Mux1/1 -> Position Blade 2/1
  Mux2/1 -> Position Blade 3/1
  Data Type Conversion/1 -> Gain/1
  Integrator/1 -> Rate Transition2/1
  Mux/1 -> Position Blade1/1
  Gain/1 -> Visualization Gain/1
  Demux/3 -> Bias2/1
  Bias/1 -> Mux/2
  Actuators/1 -> Data Type Conversion/1
  Demux/4 -> Bias3/1
  Rate Transition2/1 -> Demux/1
  Demux/1 -> Bias/1

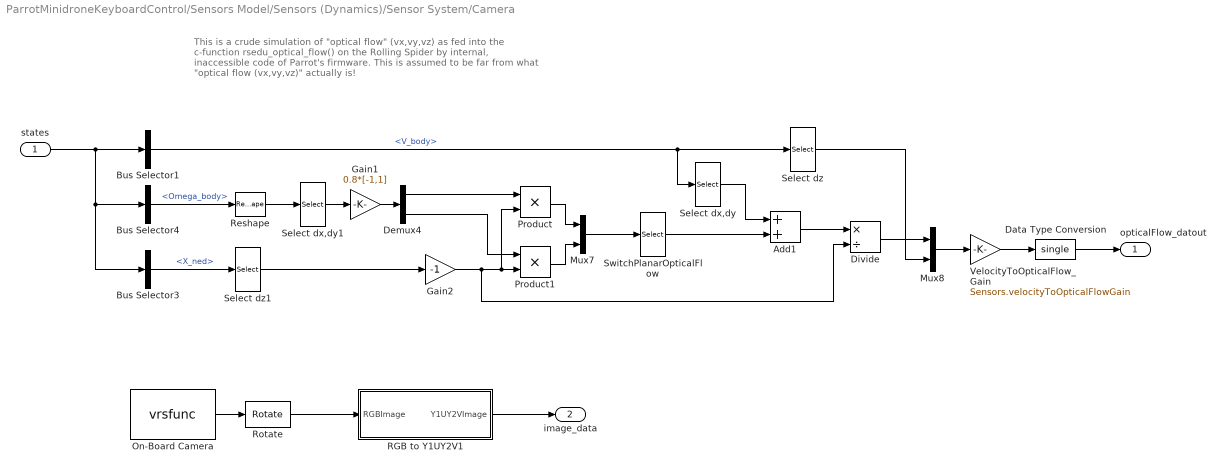
== system ParrotMinidroneKeyboardControl/Sensors Model/Sensors (Dynamics)/Sensor System/Camera ==
  note: This is a crude simulation of "optical flow" (vx,vy,vz) as
      | fed into the c-function rsedu_optical_flow() on the Rolling Spider
      | by internal, inaccessible code of Parrot's firmware.
      | This is assumed to be far from what "optical flow (vx,vy,vz)" actually is!
  states : Inport  OutDataTypeStr=Bus: StatesBus
  Add1 : Sum
  Bus Selector1 : BusSelector  OutputSignals=V_body
  Bus Selector3 : BusSelector  OutputSignals=X_ned
  Bus Selector4 : BusSelector  OutputSignals=Omega_body
  Data Type Conversion : DataTypeConversion  OutDataTypeStr=single  SaturateOnIntegerOverflow=off  RndMeth=Floor
  Demux4 : Demux  Outputs=2
  Divide : Product  Inputs=*/
  Gain1 : Gain  Gain=0.8*[-1,1]
  Gain2 : Gain  Gain=-1
  Mux7 : Mux  Inputs=2
  Mux8 : Mux  Inputs=2
  On-Board Camera : S-Function  InstantiateOnLoad=on  LoadFcn=vrmfunc('FnLoad', gcbh);  InitFcn=""  StartFcn=vrmfunc('FnSimStatus', gcbh, 'running')  StopFcn=vrmfunc('FnStop', gcbh)  FunctionName=vrsfunc  Parameters=SampleTime, VideoDimensions, false  SFunctionDeploymentMode=off  EnableBusSupport=off  mask(Virtual Reality Sink){SampleTime=VTs, ViewEnable=on, RemoteChange=off, RemoteView=off, FieldsWritten=, WorldFileName=asbQuadcopterWorld.wrl, WorldDescription=, AutoView=off, VideoDimensions=[160 120], AllowVariableSize=off, FigureProperties={'Position', 'Name', 'Viewpoint', 'CameraBound', 'CameraDirection', 'CameraPosition', 'CameraUpVector', 'ZoomFactor', 'Antialiasing', 'Headlight', 'Lighting', 'Sound', 'StatusBar', 'Stereo3D', 'Stereo3DCameraOffset', 'Stereo3DHIT', 'ToolBar', 'Textures', 'Transparency', 'Triad', 'Wireframe', 'NavZones', 'NavMode', 'NavSpeed', 'CaptureFileFormat', 'CaptureFileName', 'Record2DCompressMethod', 'Record2DCompressQuality', 'Record2D', 'Record2DFileName', 'Record2DFPS'; [5.0000000000000000e+00   9.2000000000000000e+01   5.7600000000000000e+02   3.8000000000000000e+02], 'Minidrone Flight Visualization', 'Isometric', 'on', [0.0000000000000000e+00   0.0000000000000000e+00  -1.0000000000000000e+00], [0.0000000000000000e+00   0.0000000000000000e+00   0.0000000000000000e+00], [0.0000000000000000e+00   1.0000000000000000e+00   0.0000000000000000e+00], [1.0000000000000000e+00], 'on', 'on', 'on', 'off', 'off', 'off', [1.0000000000000001e-01], [0.0000000000000000e+00], 'off', 'on', 'on', 'none', 'off', 'off', 'examine', 'normal', 'tif', '%f_anim_%n.tif', 'auto', [7.5000000000000000e+01], 'off', '***video***', 'auto'}}
      mask prompts: SampleTime "Sample Time"; ViewEnable "View"; RemoteChange "Remote Change"; RemoteView "Remote View"; FieldsWritten "Fields Written"; WorldFileName "World File Name"; WorldDescription "World Description"; VideoDimensions "Video Dimensions"; AllowVariableSize "Allow Variable Size"; FigureProperties "Figure Properties"
      mask help: Controls the selected fields of a virtual world according to given inputs.
      mask init:
      | set_param(gcbh, 'MaskDisplay', vrmfunc('FnIcon'));
      settings: CopyFcn=vrmfunc('FnCopy', gcbh);  DeleteFcn=vrmfunc('FnDelete', gcbh);  PreSaveFcn=vrmfunc('FnPreSave', gcbh);  PauseFcn=vrmfunc('FnSimStatus', gcbh, 'paused');  ContinueFcn=vrmfunc('FnSimStatus', gcbh, 'running');  DestroyFcn=vrmfunc('FnDestroy', gcbh);  OpenFcn=vrmfunc('FnOpen', gcbh);  CloseFcn=vrmfunc('FnClose', gcbh);
      mask Help: helpview(vrmfunc('FnHelpTopic'), 'vr_vrtovideo');
      mask Display: image(imread('vrblockicon.png'));
  Product : Product
  Product1 : Product
  RGB to Y1UY2V1 : Subsystem
  Reshape : Reshape
  Rotate : visiongeotforms/Rotate  outSizeR=Expanded to fit rotated input image  src_angle=Specify via dialog  unit_angle=Degrees  angle=pi/2  maxAngle=pi  dispImage=Top-left corner  method=Table lookup  fillVal=0  interpMethod=Bilinear  roundingMode=Nearest  overflowMode=on  prodOutputMode=Binary point scaling  prodOutputWordLength=32  prodOutputFracLength=10
  Select dx,dy : Selector  InputPortWidth=3  IndexOptions=Index vector (dialog)  Indices=[1 2]  OutputSizes=1
  Select dx,dy1 : Selector  InputPortWidth=3  IndexOptions=Index vector (dialog)  Indices=[1 2]  OutputSizes=1
  Select dz : Selector  InputPortWidth=3  IndexOptions=Index vector (dialog)  Indices=3  OutputSizes=1
  Select dz1 : Selector  InputPortWidth=3  IndexOptions=Index vector (dialog)  Indices=3  OutputSizes=1
  SwitchPlanarOpticalFlow : Selector  InputPortWidth=2  IndexOptions=Index vector (dialog)  Indices=[2 1]  OutputSizes=1
  VelocityToOpticalFlow_Gain : Gain  Gain=Sensors.velocityToOpticalFlowGain
  opticalFlow_datout : Outport  VectorParamsAs1DForOutWhenUnconnected=off
  image_data : Outport  Port=2  VectorParamsAs1DForOutWhenUnconnected=off
  wires:
  SwitchPlanarOpticalFlow/1 -> Add1/2
  Select dz/1 -> Mux8/2
  Bus Selector3/1 -> Select dz1/1  "<X_ned>"
  Mux7/1 -> SwitchPlanarOpticalFlow/1
  Bus Selector4/1 -> Reshape/1  "<Omega_body>"
  VelocityToOpticalFlow_Gain/1 -> Data Type Conversion/1
  Select dx,dy/1 -> Add1/1
  Reshape/1 -> Select dx,dy1/1
  Data Type Conversion/1 -> opticalFlow_datout/1
  Gain2/1 -> Divide/2, Product1/2, Product/2
  Divide/1 -> Mux8/1
  Product1/1 -> Mux7/2
  Select dx,dy1/1 -> Gain1/1
  On-Board Camera/1 -> Rotate/1
  Product/1 -> Mux7/1
  RGB to Y1UY2V1/1(Y1UY2VImage) -> image_data/1
  Demux4/1 -> Product/1
  Gain1/1 -> Demux4/1
  Select dz1/1 -> Gain2/1
  Rotate/1 -> RGB to Y1UY2V1/1(RGBImage)
  Bus Selector1/1 -> Select dz/1, Select dx,dy/1  "<V_body>"
  Demux4/2 -> Product1/1
  Mux8/1 -> VelocityToOpticalFlow_Gain/1
  states/1 -> Bus Selector1/1, Bus Selector4/1, Bus Selector3/1
  Add1/1 -> Divide/1

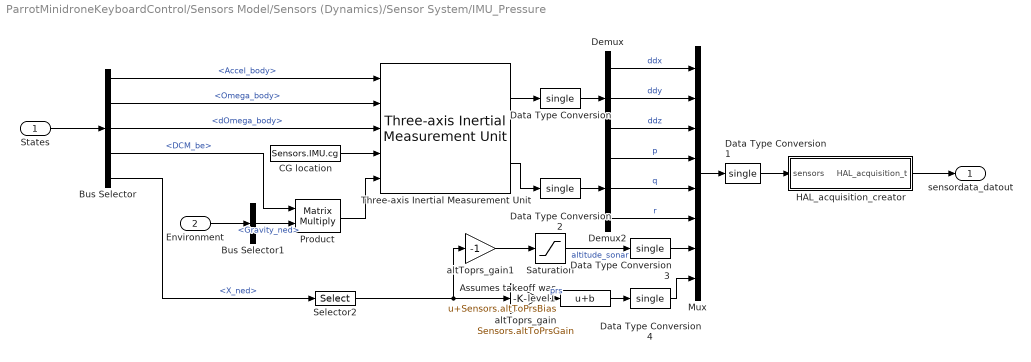
== system ParrotMinidroneKeyboardControl/Sensors Model/Sensors (Dynamics)/Sensor System/IMU_Pressure ==
  States : Inport
  Environment : Inport  Port=2
  Assumes takeoff was level1 : Bias  Bias=Sensors.altToPrsBias  SaturateOnIntegerOverflow=off
  Bus Selector : BusSelector  OutputSignals=Accel_body,Omega_body,dOmega_body,DCM_be,X_ned
  Bus Selector1 : BusSelector  OutputSignals=Gravity_ned
  CG location : Constant  Value=Sensors.IMU.cg
  Data Type Conversion{,1..4} (5 alike) : DataTypeConversion  OutDataTypeStr=single  SaturateOnIntegerOverflow=off  RndMeth=Floor
  Demux : Demux  Outputs=3
  Demux2 : Demux  Outputs=3
  HAL_acquisition_creator : Subsystem
  Mux : Mux  Inputs=8
  Product : Product  Multiplication=Matrix(*)
  Saturation : Saturate  UpperLimit=inf  LowerLimit=Sensors.altSensorMin  OutDataTypeStr=single
  Selector2 : Selector  InputPortWidth=3  IndexOptions=Index vector (dialog)  Indices=[3]  OutputSizes=1
  Three-axis Inertial Measurement Unit : aerolibnav/Three-axis Inertial Measurement Unit  units=Metric (MKS)  imu=Sensors.IMU.location  i_Ts=Ts  dtype_a=off  w_a=.7  z_a=.2  a_sf_cc=Sensors.IMU.accScaleCross  a_bias=Sensors.IMU.accBias  a_sat=Sensors.IMU.accLimits  dtype_g=off  w_g=.7  z_g=.2  g_sf_cc=Sensors.IMU.gyroScaleCross  g_bias=Sensors.IMU.gyroBias  g_sens=Sensors.IMU.gyroGBias  g_sat=Sensors.IMU.gyroLimits  i_rand=on  i_seeds=Sensors.IMU.noiseSeeds  i_pow=Sensors.IMU.noisePower
  altToprs_gain : Gain  Gain=Sensors.altToPrsGain  ParamDataTypeStr=single  OutDataTypeStr=single
  altToprs_gain1 : Gain  Gain=-1  ParamDataTypeStr=single  OutDataTypeStr=single
  sensordata_datout : Outport  OutDataTypeStr=Bus: HAL_acquisition_t  VectorParamsAs1DForOutWhenUnconnected=off
  wires:
  altToprs_gain1/1 -> Saturation/1
  Data Type Conversion4/1 -> Mux/8
  Data Type Conversion3/1 -> Mux/7
  Data Type Conversion2/1 -> Demux2/1
  Data Type Conversion/1 -> Demux/1
  Assumes takeoff was level1/1 -> Data Type Conversion4/1
  Bus Selector/5 -> Selector2/1  "<X_ned>"
  States/1 -> Bus Selector/1
  Product/1 -> Three-axis Inertial Measurement Unit/5
  Bus Selector1/1 -> Product/2  "<Gravity_ned>"
  Bus Selector/4 -> Product/1  "<DCM_be>"
  CG location/1 -> Three-axis Inertial Measurement Unit/4
  Bus Selector/3 -> Three-axis Inertial Measurement Unit/3  "<dOmega_body>"
  Environment/1 -> Bus Selector1/1
  Bus Selector/2 -> Three-axis Inertial Measurement Unit/2  "<Omega_body>"
  Bus Selector/1 -> Three-axis Inertial Measurement Unit/1  "<Accel_body>"
  HAL_acquisition_creator/1(HAL_acquisition_t) -> sensordata_datout/1
  Data Type Conversion1/1 -> HAL_acquisition_creator/1(sensors)
  Three-axis Inertial Measurement Unit/2 -> Data Type Conversion2/1
  Three-axis Inertial Measurement Unit/1 -> Data Type Conversion/1
  Mux/1 -> Data Type Conversion1/1
  altToprs_gain/1 -> Assumes takeoff was level1/1  "prs"
  Saturation/1 -> Data Type Conversion3/1  "altitude_sonar"
  Selector2/1 -> altToprs_gain/1, altToprs_gain1/1
  Demux/3 -> Mux/3  "ddz"
  Demux2/3 -> Mux/6  "r"
  Demux/2 -> Mux/2  "ddy"
  Demux/1 -> Mux/1  "ddx"
  Demux2/1 -> Mux/4  "p"
  Demux2/2 -> Mux/5  "q"

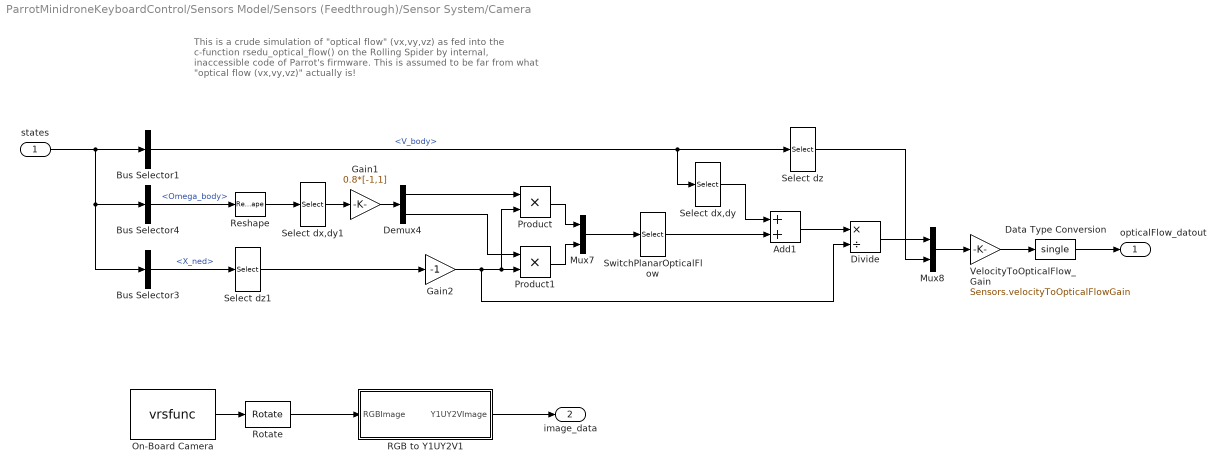
== system ParrotMinidroneKeyboardControl/Sensors Model/Sensors (Feedthrough)/Sensor System/Camera ==
  note: This is a crude simulation of "optical flow" (vx,vy,vz) as
      | fed into the c-function rsedu_optical_flow() on the Rolling Spider
      | by internal, inaccessible code of Parrot's firmware.
      | This is assumed to be far from what "optical flow (vx,vy,vz)" actually is!
  states : Inport  OutDataTypeStr=Bus: StatesBus
  Add1 : Sum
  Bus Selector1 : BusSelector  OutputSignals=V_body
  Bus Selector3 : BusSelector  OutputSignals=X_ned
  Bus Selector4 : BusSelector  OutputSignals=Omega_body
  Data Type Conversion : DataTypeConversion  OutDataTypeStr=single  SaturateOnIntegerOverflow=off  RndMeth=Floor
  Demux4 : Demux  Outputs=2
  Divide : Product  Inputs=*/
  Gain1 : Gain  Gain=0.8*[-1,1]
  Gain2 : Gain  Gain=-1
  Mux7 : Mux  Inputs=2
  Mux8 : Mux  Inputs=2
  On-Board Camera : S-Function  InstantiateOnLoad=on  LoadFcn=vrmfunc('FnLoad', gcbh);  InitFcn=""  StartFcn=vrmfunc('FnSimStatus', gcbh, 'running')  StopFcn=vrmfunc('FnStop', gcbh)  FunctionName=vrsfunc  Parameters=SampleTime, VideoDimensions, false  SFunctionDeploymentMode=off  EnableBusSupport=off  mask(Virtual Reality Sink){SampleTime=VTs, ViewEnable=on, RemoteChange=off, RemoteView=off, FieldsWritten=, WorldFileName=asbQuadcopterWorld.wrl, WorldDescription=, AutoView=off, VideoDimensions=[160 120], AllowVariableSize=off, FigureProperties=[]}
      mask prompts: SampleTime "Sample Time"; ViewEnable "View"; RemoteChange "Remote Change"; RemoteView "Remote View"; FieldsWritten "Fields Written"; WorldFileName "World File Name"; WorldDescription "World Description"; VideoDimensions "Video Dimensions"; AllowVariableSize "Allow Variable Size"; FigureProperties "Figure Properties"
      mask help: Controls the selected fields of a virtual world according to given inputs.
      mask init:
      | set_param(gcbh, 'MaskDisplay', vrmfunc('FnIcon'));
      settings: CopyFcn=vrmfunc('FnCopy', gcbh);  DeleteFcn=vrmfunc('FnDelete', gcbh);  PreSaveFcn=vrmfunc('FnPreSave', gcbh);  PauseFcn=vrmfunc('FnSimStatus', gcbh, 'paused');  ContinueFcn=vrmfunc('FnSimStatus', gcbh, 'running');  DestroyFcn=vrmfunc('FnDestroy', gcbh);  OpenFcn=vrmfunc('FnOpen', gcbh);  CloseFcn=vrmfunc('FnClose', gcbh);
      mask Help: helpview(vrmfunc('FnHelpTopic'), 'vr_vrtovideo');
      mask Display: image(imread('vrblockicon.png'));
  Product : Product
  Product1 : Product
  RGB to Y1UY2V1 : Subsystem
  Reshape : Reshape
  Rotate : visiongeotforms/Rotate  outSizeR=Expanded to fit rotated input image  src_angle=Specify via dialog  unit_angle=Degrees  angle=pi/2  maxAngle=pi  dispImage=Top-left corner  method=Table lookup  fillVal=0  interpMethod=Bilinear  roundingMode=Nearest  overflowMode=on  prodOutputMode=Binary point scaling  prodOutputWordLength=32  prodOutputFracLength=10
  Select dx,dy : Selector  InputPortWidth=3  IndexOptions=Index vector (dialog)  Indices=[1 2]  OutputSizes=1
  Select dx,dy1 : Selector  InputPortWidth=3  IndexOptions=Index vector (dialog)  Indices=[1 2]  OutputSizes=1
  Select dz : Selector  InputPortWidth=3  IndexOptions=Index vector (dialog)  Indices=3  OutputSizes=1
  Select dz1 : Selector  InputPortWidth=3  IndexOptions=Index vector (dialog)  Indices=3  OutputSizes=1
  SwitchPlanarOpticalFlow : Selector  InputPortWidth=2  IndexOptions=Index vector (dialog)  Indices=[2 1]  OutputSizes=1
  VelocityToOpticalFlow_Gain : Gain  Gain=Sensors.velocityToOpticalFlowGain
  opticalFlow_datout : Outport  VectorParamsAs1DForOutWhenUnconnected=off
  image_data : Outport  Port=2  VectorParamsAs1DForOutWhenUnconnected=off
  wires:
  states/1 -> Bus Selector1/1, Bus Selector4/1, Bus Selector3/1
  Demux4/2 -> Product1/1
  Demux4/1 -> Product/1
  Bus Selector1/1 -> Select dz/1, Select dx,dy/1  "<V_body>"
  Rotate/1 -> RGB to Y1UY2V1/1(RGBImage)
  Gain1/1 -> Demux4/1
  Add1/1 -> Divide/1
  Product/1 -> Mux7/1
  Select dz1/1 -> Gain2/1
  On-Board Camera/1 -> Rotate/1
  Select dx,dy1/1 -> Gain1/1
  Gain2/1 -> Divide/2, Product1/2, Product/2
  Reshape/1 -> Select dx,dy1/1
  Divide/1 -> Mux8/1
  Data Type Conversion/1 -> opticalFlow_datout/1
  RGB to Y1UY2V1/1(Y1UY2VImage) -> image_data/1
  VelocityToOpticalFlow_Gain/1 -> Data Type Conversion/1
  Product1/1 -> Mux7/2
  Mux7/1 -> SwitchPlanarOpticalFlow/1
  Mux8/1 -> VelocityToOpticalFlow_Gain/1
  Select dx,dy/1 -> Add1/1
  Bus Selector4/1 -> Reshape/1  "<Omega_body>"
  Select dz/1 -> Mux8/2
  Bus Selector3/1 -> Select dz1/1  "<X_ned>"
  SwitchPlanarOpticalFlow/1 -> Add1/2

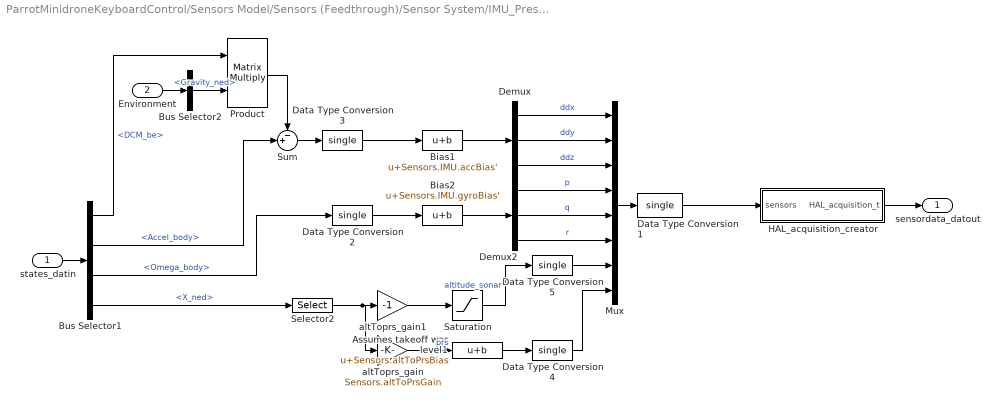
== system ParrotMinidroneKeyboardControl/Sensors Model/Sensors (Feedthrough)/Sensor System/IMU_Pressure ==
  states_datin : Inport  OutDataTypeStr=Bus: StatesBus
  Environment : Inport  Port=2
  Assumes takeoff was level1 : Bias  Bias=Sensors.altToPrsBias  SaturateOnIntegerOverflow=off
  Bias1 : Bias  Bias=Sensors.IMU.accBias'  SaturateOnIntegerOverflow=off
  Bias2 : Bias  Bias=Sensors.IMU.gyroBias'  SaturateOnIntegerOverflow=off
  Bus Selector1 : BusSelector  OutputSignals=DCM_be,Accel_body,Omega_body,X_ned
  Bus Selector2 : BusSelector  OutputSignals=Gravity_ned
  Data Type Conversion{1..5} (5 alike) : DataTypeConversion  OutDataTypeStr=single  SaturateOnIntegerOverflow=off  RndMeth=Floor
  Demux : Demux  Outputs=3
  Demux2 : Demux  Outputs=3
  HAL_acquisition_creator : Subsystem
  Mux : Mux  Inputs=8
  Product : Product  Multiplication=Matrix(*)
  Saturation : Saturate  UpperLimit=inf  LowerLimit=Sensors.altSensorMin  OutDataTypeStr=single
  Selector2 : Selector  InputPortWidth=3  IndexOptions=Index vector (dialog)  Indices=[3]  OutputSizes=1
  Sum : Sum  Inputs=-+|
  altToprs_gain : Gain  Gain=Sensors.altToPrsGain  ParamDataTypeStr=single  OutDataTypeStr=single
  altToprs_gain1 : Gain  Gain=-1  ParamDataTypeStr=single  OutDataTypeStr=single
  sensordata_datout : Outport  OutDataTypeStr=Bus: HAL_acquisition_t  VectorParamsAs1DForOutWhenUnconnected=off
  wires:
  Bias2/1 -> Demux2/1
  Bias1/1 -> Demux/1
  Product/1 -> Sum/1
  Bus Selector1/2 -> Sum/2  "<Accel_body>"
  Sum/1 -> Data Type Conversion3/1
  Bus Selector1/1 -> Product/1  "<DCM_be>"
  Bus Selector2/1 -> Product/2  "<Gravity_ned>"
  altToprs_gain1/1 -> Saturation/1
  Data Type Conversion5/1 -> Mux/7
  Data Type Conversion4/1 -> Mux/8
  Data Type Conversion2/1 -> Bias2/1
  Data Type Conversion3/1 -> Bias1/1
  Assumes takeoff was level1/1 -> Data Type Conversion4/1
  Bus Selector1/4 -> Selector2/1  "<X_ned>"
  states_datin/1 -> Bus Selector1/1
  Environment/1 -> Bus Selector2/1
  Bus Selector1/3 -> Data Type Conversion2/1  "<Omega_body>"
  HAL_acquisition_creator/1(HAL_acquisition_t) -> sensordata_datout/1
  Data Type Conversion1/1 -> HAL_acquisition_creator/1(sensors)
  Mux/1 -> Data Type Conversion1/1
  altToprs_gain/1 -> Assumes takeoff was level1/1  "prs"
  Saturation/1 -> Data Type Conversion5/1  "altitude_sonar"
  Selector2/1 -> altToprs_gain1/1, altToprs_gain/1
  Demux/3 -> Mux/3  "ddz"
  Demux2/3 -> Mux/6  "r"
  Demux/2 -> Mux/2  "ddy"
  Demux/1 -> Mux/1  "ddx"
  Demux2/1 -> Mux/4  "p"
  Demux2/2 -> Mux/5  "q"
